simulink model "induction_machine_skalarne"  (R2026b)
settings: Solver=FixedStepAuto  StopTime=10  FixedStep=Ts
PreLoadFcn:
  | Ts = 250e-6;
InitFcn:
  | Ts = 250e-6;
libraries: autolibim x1, SignalEditorBlockLib x1
settings Model: Creator=Kajo  LastModifiedBy=patrikmitro

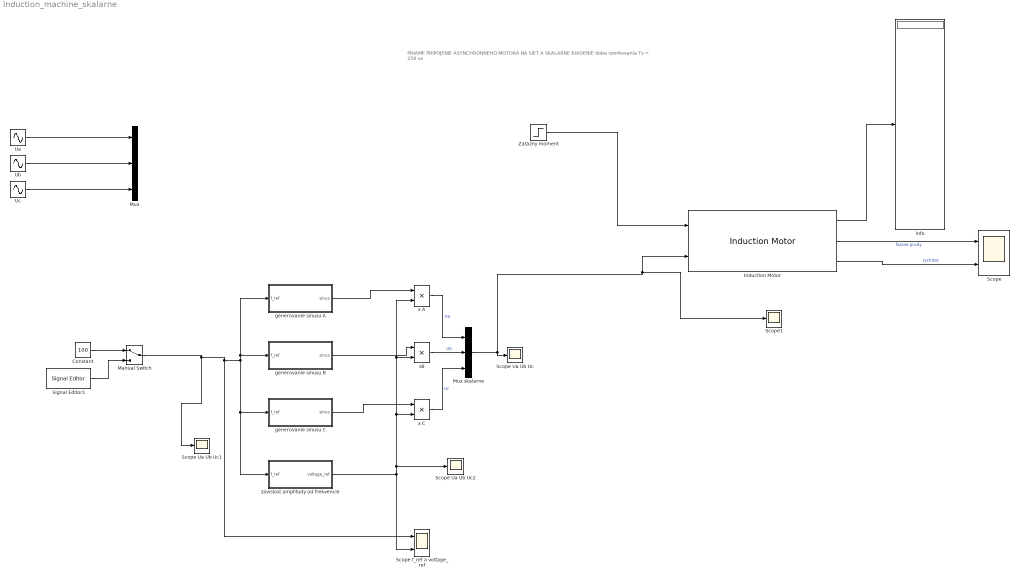
== system induction_machine_skalarne ==
  note: PRIAME PRIPOJENIE ASYNCHRONNEHO MOTORA NA SIET A SKALARNE RIADENIE
      | doba vzorkovania Ts = 250 us
  Constant : Constant  Value=100
  Induction Motor : autolibim/Induction Motor  sim_type=Continuous  Ts=0.001  port_config=Torque  P=1  Zs=[4.36 0.013]  Zr="[2.16  0.013]"  Lm=0.46  mechanical=[0.0017 0.001 0]  theta_init=0  omega_init=0  RefBlkName='autolibim/Induction Motor'  aMode=5
      settings: LibrarySourceBlock=mcblib/Control/Induction Machine/Electrical Systems/Motors/Induction Motor
  Manual Switch : ManualSwitch
  Mux : Mux  Inputs=3
  Mux skalarne : Mux  Inputs=3
  Scope : Scope  NumInputPorts=2
      settings: ActiveDisplayYMinimum=-47.012341582832107  ActiveDisplayYMaximum=50.829584514722512
  Scope Ua Ub Uc : Scope
  Scope Ua Ub Uc1 : Scope
      settings: ActiveDisplayYMinimum=-12.499999999999996  ActiveDisplayYMaximum=112.5  DataLoggingVariableName=ScopeData2
  Scope Ua Ub Uc2 : Scope
      settings: ActiveDisplayYMinimum=-21.849999999999994  ActiveDisplayYMaximum=424.65  DataLoggingVariableName=ScopeData3
  Scope f_ref a voltage_ref : Scope  NumInputPorts=2
      settings: ActiveDisplayYMinimum=18.811109688092856  ActiveDisplayYMaximum=25.560982165119594
  Scope1 : Scope
      settings: ActiveDisplayYMinimum=-475  ActiveDisplayYMaximum=475
  Signal Editor1 : SignalEditorBlockLib/Signal Editor  FileName=untitled.mat  ActiveScenario=Scenario  ActiveSignal=Signal 1  IsBus=off  OutputBusObjectStr=Bus: BusObject  SampleTime=0  ZeroCross=off  OutputAfterFinalValue=Setting to zero  Unit=inherit  PreserveSignalName=on  ApplySigPropsToAllScenarios=off  ApplySigPropsToAllSignals=off  SignalPropertySource=Signal data in MAT file
  Ua : Sin  Amplitude=380  Frequency=2*pi*50  SampleTime=0
  Ub : Sin  Amplitude=380  Frequency=2*pi*50  Phase=-(2*pi)/3  SampleTime=0
  Uc : Sin  Amplitude=380  Frequency=2*pi*50  Phase=-(4*pi)/3  SampleTime=0
  Zatazny moment : Step  Time=2  FinalValue=4.98  SampleTime=0
  generovanie sinusu A : Subsystem
  generovanie sinusu B : Subsystem
  generovanie sinusu C : Subsystem
  info : Display
  sB : Product
  x A : Product
  x C : Product
  zavislost amplitudy od frekvencie : MATLAB Function  TreatAsAtomicUnit=on
  wires:
  Ua/1 -> Mux/1
  Ub/1 -> Mux/2
  Uc/1 -> Mux/3
  Zatazny moment/1 -> Induction Motor/1
  Induction Motor/2 -> Scope/1  "fazove prudy"
  Induction Motor/3 -> Scope/2  "rychlost"
  Induction Motor/1 -> info/1
  Manual Switch/1 -> Scope Ua Ub Uc1/1, Scope f_ref a voltage_ref/1, generovanie sinusu C/1(f_ref), zavislost amplitudy od frekvencie/1(f_ref), generovanie sinusu A/1(f_ref), generovanie sinusu B/1(f_ref)
  zavislost amplitudy od frekvencie/1(voltage_ref) -> Scope Ua Ub Uc2/1, x A/2, sB/2, x C/2, Scope f_ref a voltage_ref/2
  generovanie sinusu A/1(sinus) -> x A/1
  x A/1 -> Mux skalarne/1  "Ua"
  generovanie sinusu B/1(sinus) -> sB/1
  sB/1 -> Mux skalarne/2  "Ub"
  generovanie sinusu C/1(sinus) -> x C/1
  x C/1 -> Mux skalarne/3  "Uc"
  Mux skalarne/1 -> Induction Motor/2, Scope1/1, Scope Ua Ub Uc/1
  Constant/1 -> Manual Switch/1
  Signal Editor1/1 -> Manual Switch/2

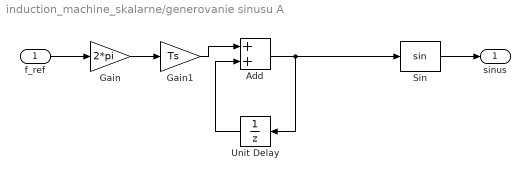
== system induction_machine_skalarne/generovanie sinusu A ==
  f_ref : Inport
  Add : Sum
  Gain : Gain  Gain=2*pi
  Gain1 : Gain  Gain=Ts
  Sin : Trigonometry
  Unit Delay : UnitDelay  SampleTime=Ts
  sinus : Outport
  wires:
  f_ref/1 -> Gain/1
  Gain/1 -> Gain1/1
  Gain1/1 -> Add/1
  Add/1 -> Unit Delay/1, Sin/1
  Unit Delay/1 -> Add/2
  Sin/1 -> sinus/1

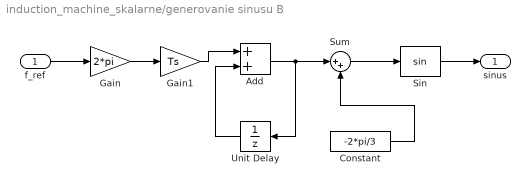
== system induction_machine_skalarne/generovanie sinusu B ==
  f_ref : Inport
  Add : Sum
  Constant : Constant  Value=-2*pi/3
  Gain : Gain  Gain=2*pi
  Gain1 : Gain  Gain=Ts
  Sin : Trigonometry
  Sum : Sum  Inputs=|++
  Unit Delay : UnitDelay  SampleTime=Ts
  sinus : Outport
  wires:
  f_ref/1 -> Gain/1
  Gain/1 -> Gain1/1
  Gain1/1 -> Add/1
  Add/1 -> Unit Delay/1, Sum/1
  Unit Delay/1 -> Add/2
  Constant/1 -> Sum/2
  Sum/1 -> Sin/1
  Sin/1 -> sinus/1

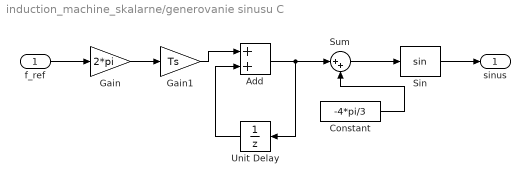
== system induction_machine_skalarne/generovanie sinusu C ==
  f_ref : Inport
  Add : Sum
  Constant : Constant  Value=-4*pi/3
  Gain : Gain  Gain=2*pi
  Gain1 : Gain  Gain=Ts
  Sin : Trigonometry
  Sum : Sum  Inputs=|++
  Unit Delay : UnitDelay  SampleTime=Ts
  sinus : Outport
  wires:
  f_ref/1 -> Gain/1
  Gain/1 -> Gain1/1
  Gain1/1 -> Add/1
  Add/1 -> Unit Delay/1, Sum/1
  Unit Delay/1 -> Add/2
  Constant/1 -> Sum/2
  Sum/1 -> Sin/1
  Sin/1 -> sinus/1

== matlab function induction_machine_skalarne/zavislost amplitudy od frekvencie ==
  data: f_ref input; voltage_ref output
function voltage_ref = fcn(f_ref)
% Zavislost amplitudy fazoveho napatia od frekvencie (obr. 1)
Un     = 380;          % amplituda napatia pri menovitej frekvencii [V]
fn     = 50;           % menovita frekvencia [Hz]
fb     = 3;            % hranica oblasti Uboost [Hz]
Uboost = Un/fn*fb;     % konstantne napatie pre 0..3 Hz (22,8 V)

if f_ref < 0
    voltage_ref = 0;               % f < 0 Hz: neplatna frekvencia
elseif f_ref <= fb
    voltage_ref = Uboost;          % 0..3 Hz: Uboost
elseif f_ref <= fn
    voltage_ref = Un/fn*f_ref;     % 3..50 Hz: U/f = konst.
else
    voltage_ref = Un;              % f > 50 Hz: napatie sa uz nezvysuje
end
end
